simulink model "model_23b"  (R2023b)
settings: Solver=ode45  StartTime=TSPAN(1)  StopTime=TSPAN(2)  MaxStep=MaxStep  RelTol=RelTol  AbsTol=AbsTol
values from neighbouring files (symbols this model uses):
  cal_V0_ini = 0    [init.m]
  dim_xp = numel(xp_0)    [init.m]
  JSPAN = [0 30*TSPAN(2)]    [init.m]
  parameters = struct()    [init.m]
  TSPAN = [0 300]    [init.m]
  xc_0 = [chi_0;theta_0]    [init.m]
  xp_0 = [p_0;q_0;v_0;o_0]    [init.m]
libraries: HyEQ_Library x6
(part 2 of 2)

== matlab function model_23b/MATLAB Function9 ==
  data: xp input; value_a output; xc input; parameters parameter
function value_a = fcn(xp,xc,parameters)

x0=[xp;xc];

value_a=a(x0,parameters);

end

== matlab function model_23b/output eqn of H (safe)1 ==
  data: xp input; control output; xc input; parameters parameter
function control = fcn(xp,xc,parameters)

x0=[xp;xc];

control=kappa_2(x0,parameters);

end

== matlab function model_23b/plant2 ==
  data: xp input; dxp output; control input; parameters parameter
function dxp = fcn(xp,control,parameters)

dxp=f_p(xp,control,parameters);

end

== matlab function model_23b/Hybrid System with Input2/flow map f ==
  data: state input size=state_dim; xp input size=input_dim; dstate output size=state_dim; parameters parameter
function dstate = f(state, xp, parameters)

dstate=f_flow(state, xp, parameters);

end

== matlab function model_23b/Hybrid System with Input2/flow set C ==
  data: state input size=state_dim; xp input size=input_dim; inC output size=1; parameters parameter
function inC = C(state, xp, parameters)
   inC=1;
end

== matlab function model_23b/Hybrid System with Input2/jump map g ==
  data: state input size=state_dim; xp input size=input_dim; nextstate output size=state_dim; parameters parameter
function nextstate = g(state, xp, parameters)

nextstate=f_jump(state, xp, parameters);

end

== matlab function model_23b/Hybrid System with Input1/flow map f ==
  data: state input size=state_dim; xp input size=input_dim; dstate output size=state_dim; parameters parameter
function dstate = f(state, xp, parameters)

xc=state(1:3);
cal_V0=state(4);

x0=[xp;xc];

dxc=f_flow(xc, xp, parameters);
cal_dV0=fcn_dV0(x0,parameters);

dstate=[dxc;cal_dV0];

end

== matlab function model_23b/Hybrid System with Input2/jump set D ==
  data: state input size=state_dim; xp input size=input_dim; inD output size=1; parameters parameter
function inD = D(state, xp, parameters)
   inD=0;
end

== matlab function model_23b/Hybrid System with Input3/flow map f ==
  data: state input size=state_dim; xp input size=input_dim; dstate output size=state_dim; parameters parameter
function dstate = f(state, xp, parameters)

xc=state(1:3);
cal_V0=state(4);

x0=[xp;xc];

dxc=f_flow(xc, xp, parameters);
cal_dV0=fcn_dV0(x0,parameters);

dstate=[dxc;cal_dV0];

end

== matlab function model_23b/Hybrid System with Input3/flow set C ==
  data: state input size=state_dim; xp input size=input_dim; inC output size=1; parameters parameter
function inC = C(state, xp, parameters)

    xc=state(1:3);

   [inC,~]=fcn_decide(xc,xp,parameters);
end

== matlab function model_23b/Hybrid System with Input3/jump map g ==
  data: state input size=state_dim; xp input size=input_dim; nextstate output size=state_dim; parameters parameter
function nextstate = g(state, xp, parameters)

delta=parameters.delta;

xc=state(1:3);
cal_V0=state(4);


nextxc=f_jump(state, xp, parameters);
cal_nextV0=cal_V0-delta;

nextstate=[nextxc;cal_nextV0];

end

== matlab function model_23b/Hybrid System with Input3/jump set D ==
  data: state input size=state_dim; xp input size=input_dim; inD output size=1; parameters parameter
function inD = D(state, xp, parameters)

xc=state(1:3);
   [~,inD]=fcn_decide(xc,xp,parameters);
end

== matlab function model_23b/Lya3 ==
  data: xp input; V0 output; xc input; parameters parameter
function V0 = fcn(xp,xc,parameters)

x0=[xp;xc];

V0=fcn_V0(x0,parameters);

end

== matlab function model_23b/MATLAB Function12 ==
  data: xp input; xc input; min_Lya output; parameters parameter
function min_Lya = fcn(xp,xc,parameters)

%%%
chi=xc(1:2);
% theta=state(3);

%%%
x0_0=[xp;chi;0];%theta=0
x0_1=[xp;chi;1];%theta=1
V0_0=fcn_V0(x0_0,parameters);%theta=0
V0_1=fcn_V0(x0_1,parameters);%theta=1

min_Lya=min(V0_0,V0_1);

end

== matlab function model_23b/MATLAB Function13 ==
  data: xp input; value_a output; xc input; parameters parameter
function value_a = fcn(xp,xc,parameters)

x0=[xp;xc];

value_a=a(x0,parameters);

end

== matlab function model_23b/MATLAB Function14 ==
  data: xp input; value_vartheta1 output; xc input; parameters parameter
function value_vartheta1 = fcn(xp,xc,parameters)

x0=[xp;xc];

value_vartheta1=vartheta1(x0,parameters);

end

== matlab function model_23b/MATLAB Function15 ==
  data: u input; y output
function y = fcn(u)

y = log(u+eps);

== matlab function model_23b/Hybrid System with Input/flow map f ==
  data: state input size=state_dim; xp input size=input_dim; dstate output size=state_dim; parameters parameter
function dstate = f(state, xp, parameters)

dstate=f_flow(state, xp, parameters);

end

== matlab function model_23b/compare1 ==
  data: real_V0 input; err_real_cal_V0 output; cal_V0 input; parameters parameter
function err_real_cal_V0 = fcn(real_V0,cal_V0,parameters)

persistent real_V0_ini

if isempty(real_V0_ini)
    real_V0_ini=real_V0;
end


err_real_cal_V0=log(abs(cal_V0-(real_V0-real_V0_ini))+eps);%should set cal_V0(0)=0 in the integrator


end

== matlab function model_23b/output eqn of H1 ==
  data: xp input; control output; xc input; parameters parameter
function control = fcn(xp,xc,parameters)

x0=[xp;xc];

control=kappa_0(x0,parameters);

end

== matlab function model_23b/plant3 ==
  data: xp input; dxp output; control input; parameters parameter
function dxp = fcn(xp,control,parameters)

dxp=f_p(xp,control,parameters);

end

== matlab function model_23b/Hybrid System with Input/flow set C ==
  data: state input size=state_dim; xp input size=input_dim; inC output size=1; parameters parameter
function inC = C(state, xp, parameters)
   [inC,~]=fcn_decide(state,xp,parameters);
end

== matlab function model_23b/Hybrid System with Input/jump map g ==
  data: state input size=state_dim; xp input size=input_dim; nextstate output size=state_dim; parameters parameter
function nextstate = g(state, xp, parameters)

nextstate=f_jump(state, xp, parameters);

end

== matlab function model_23b/Hybrid System with Input/jump set D ==
  data: state input size=state_dim; xp input size=input_dim; inD output size=1; parameters parameter
function inD = D(state, xp, parameters)
   [~,inD]=fcn_decide(state,xp,parameters);
end

== matlab function model_23b/compare ==
  data: real_V0 input; err_real_cal_V0 output; cal_V0 input; parameters parameter
function err_real_cal_V0 = fcn(real_V0,cal_V0,parameters)

persistent real_V0_ini

if isempty(real_V0_ini)
    real_V0_ini=real_V0;
end


err_real_cal_V0=log(abs(cal_V0-(real_V0-real_V0_ini))+eps);%should set cal_V0(0)=0 in the integrator


end

== matlab function model_23b/MATLAB Function ==
  data: xp input; xc input; min_Lya output; parameters parameter
function min_Lya = fcn(xp,xc,parameters)

%%%
chi=xc(1:2);
% theta=state(3);

%%%
x0_0=[xp;chi;0];%theta=0
x0_1=[xp;chi;1];%theta=1
V0_0=fcn_V0(x0_0,parameters);%theta=0
V0_1=fcn_V0(x0_1,parameters);%theta=1

min_Lya=min(V0_0,V0_1);

end
